simulink model "SEDC_Motor"  (R2023b)
settings: Solver=VariableStepAuto  StartTime=0.0  StopTime=0.1  MaxStep=1e-4  RelTol=1e-3
libraries: spsThyristorLib x4, spsVoltageMeasurementLib x3, spsACVoltageSourceLib x1, dspswit3 x1, spsSeriesRLCBranchLib x1, spsUniversalBridgeLib x1, sps_lib x1
settings Model: Creator=SEIF  LastModifiedBy=SEIF

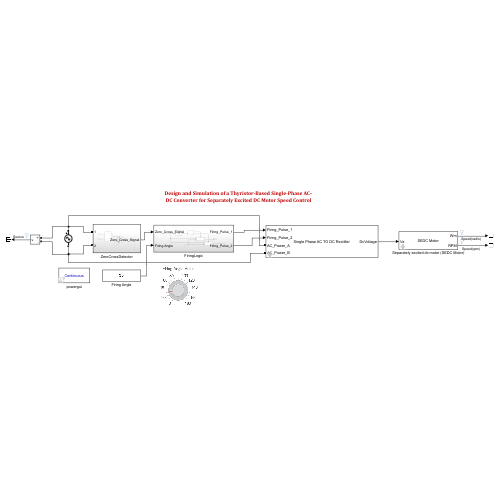
[thumbnail: Simulink's stored preview of the top-level diagram]
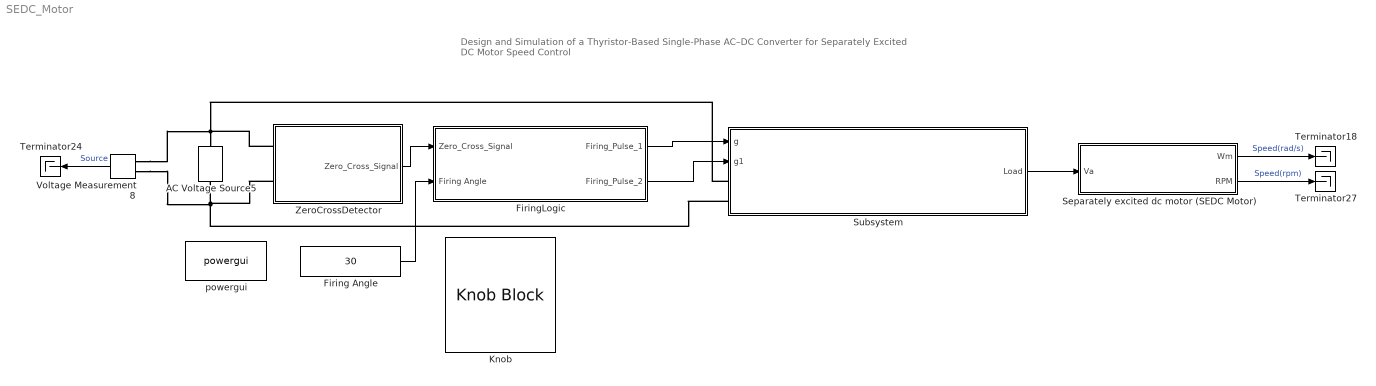
== system SEDC_Motor ==
  note: Design and Simulation of a Thyristor-Based Single-Phase AC–DC Converter for Separately Excited DC Motor Speed Control
  AC Voltage Source5 : spsACVoltageSourceLib/AC Voltage Source  Amplitude=sqrt(2) * 220  Phase=0  Frequency=50  SampleTime=0  Measurements=None  BusType=swing  Pref=10e3  Qref=0  Qmin=-inf  Qmax=+inf
  Firing Angle : Constant  Value=30
  FiringLogic : Subsystem
  Knob : KnobBlock  ScaleMax=180
  Separately excited dc motor (SEDC Motor) : Subsystem  mask{Ra=50, La=0.15, J=0.05, B=0.005, Kt=1.15, Kphi=1.15, TL=5}
      mask prompts: Ra "Armature Resistance"; La "Armature Inductance"; J "Moment of Inertia"; B "Viscous Friction"; Kt "Torque Constant"; Kphi "Back EMF Constant"; TL "Load Torque"
      mask Display:
      | disp('SEDC Motor');
      | 
      | port_label('input',1,'Va');
      | port_label('output',1,'Wm');
      | port_label('output',2,'RPM');
  Subsystem : Subsystem
      mask Display:
      | disp('Single Phase AC TO DC Rectifier');
      | 
      | port_label('input',1,'Firing_Pulse_1');
      | port_label('input',2,'Firing_Pulse_2');
      | port_label('lconn',1,'AC_Power_A');
      | port_label('lconn',2,'AC_Power_B');
      | port_label('output',1,'DcVoltage');
  Terminator18 : Terminator
  Terminator24 : Terminator
  Terminator27 : Terminator
  Voltage Measurement8 : spsVoltageMeasurementLib/Voltage Measurement  PhasorSimulation=off  OutputType=Complex  PSBequivalent=0
  ZeroCrossDetector : Subsystem
  powergui : sps_lib/powergui  Priority=1  SimulationMode=Continuous  SampleTime=50e-6  frequency=60  Iterations=50  frequencyindice=50  Pbase=100e6  ErrMax=1e-4  UnitsV=kV  UnitsW=MW  buscounter=0  FunctionMessages=off  echomessages=off  EnableUseOfTLC=off  CurrentSourceSwitches=off  DisableSnubberDevices=off  DisableRonSwitches=off  DisableVfSwitches=off  DisplayEquations=off  AutomaticDiscreteSolvers=off  SolverType=Tustin/Backward Euler (TBE)  Interpol=off  ExternalGateDelay=off  methode=off  Ts=100  x0status=blocks  SPID=on  SwTol=0  HookPort=off  NonlinearTolerance=1e-4  nMaxIteration=100  ContinueOnMaxIteration=off  RestoreLinks=warning  ResistiveCurrentMeasurement=off  Frange=[0:2:500]  Ylog=off  Xlog=on  ShowGrid=off  save=off  variable=ZData  structure=0  ZoomFFT=off  StartTime=0.0  cycles=1  DisplayStyle=1  fundamental=60  FreqAxis=off  MaxFrequency=1000  frequencyindicesteady=1  RmsSteady=1  display=off
  wires:
  Separately excited dc motor (SEDC Motor)/1(Wm) -> Terminator18/1  "Speed(rad/s)"
  ZeroCrossDetector/1(Zero_Cross_Signal) -> FiringLogic/1(Zero_Cross_Signal)
  Separately excited dc motor (SEDC Motor)/2(RPM) -> Terminator27/1  "Speed(rpm)"
  Voltage Measurement8/1 -> Terminator24/1  "Source"
  Firing Angle/1 -> FiringLogic/2(Firing Angle)
  Subsystem/1(Load) -> Separately excited dc motor (SEDC Motor)/1(Va)
  FiringLogic/1(Firing_Pulse_1) -> Subsystem/1(g)
  FiringLogic/2(Firing_Pulse_2) -> Subsystem/2(g1)
  connections:
  Voltage Measurement8/LConn2 -- Subsystem/LConn2 -- ZeroCrossDetector/LConn2 -- AC Voltage Source5/LConn1
  Voltage Measurement8/LConn1 -- Subsystem/LConn1 -- ZeroCrossDetector/LConn1 -- AC Voltage Source5/RConn1

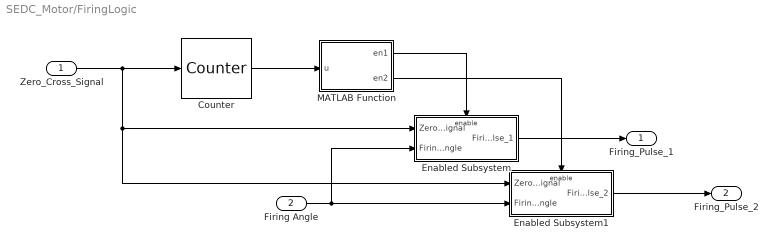
== system SEDC_Motor/FiringLogic ==
  Zero_Cross_Signal : Inport
  Firing Angle : Inport  Port=2
  Counter : dspswit3/Counter  Direction=Up  CountEvent=Rising edge  CounterSize=User defined  MaxCount=255  InitialCount=0  Output=Count  HitValue=32  ResetInput=off  SamplesPerFrame=1  Ts=1  CntDtype=double  HitDtype=Logical
  Enabled Subsystem : Subsystem  TreatAsAtomicUnit=on
  Enabled Subsystem1 : Subsystem  TreatAsAtomicUnit=on
  MATLAB Function : MATLAB Function  TreatAsAtomicUnit=on
  Firing_Pulse_1 : Outport
  Firing_Pulse_2 : Outport  Port=2
  wires:
  Zero_Cross_Signal/1 -> Enabled Subsystem1/1(Zero_Cross_Signal), Enabled Subsystem/1(Zero_Cross_Signal), Counter/1
  Counter/1 -> MATLAB Function/1(u)
  Firing Angle/1 -> Enabled Subsystem1/2(Firing Angle), Enabled Subsystem/2(Firing Angle)
  Enabled Subsystem/1(Firing_Pulse_1) -> Firing_Pulse_1/1
  Enabled Subsystem1/1(Firing_Pulse_2) -> Firing_Pulse_2/1
  MATLAB Function/1(en1) -> Enabled Subsystem/Enable
  MATLAB Function/2(en2) -> Enabled Subsystem1/Enable

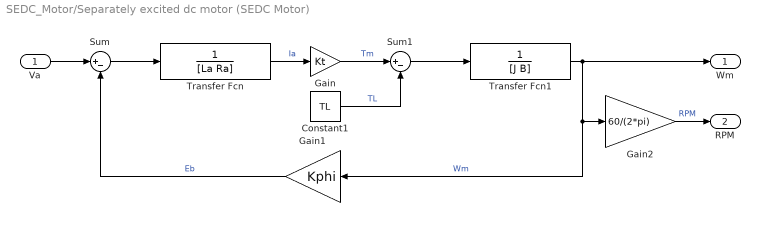
== system SEDC_Motor/Separately excited dc motor (SEDC Motor) ==
  Va : Inport
  Constant1 : Constant  Value=TL
  Gain : Gain  Gain=Kt
  Gain1 : Gain  Gain=Kphi
  Gain2 : Gain  Gain=60/(2*pi)
  Sum : Sum  Inputs=|+-
  Sum1 : Sum  Inputs=|+-
  Transfer Fcn : TransferFcn  Denominator=[La Ra]
  Transfer Fcn1 : TransferFcn  Denominator=[J B]
  Wm : Outport
  RPM : Outport  Port=2
  wires:
  Sum/1 -> Transfer Fcn/1
  Va/1 -> Sum/1
  Gain1/1 -> Sum/2  "Eb"
  Transfer Fcn/1 -> Gain/1  "Ia"
  Gain/1 -> Sum1/1  "Tm"
  Constant1/1 -> Sum1/2  "TL"
  Sum1/1 -> Transfer Fcn1/1
  Transfer Fcn1/1 -> Gain1/1, Gain2/1, Wm/1  "Wm"
  Gain2/1 -> RPM/1  "RPM"

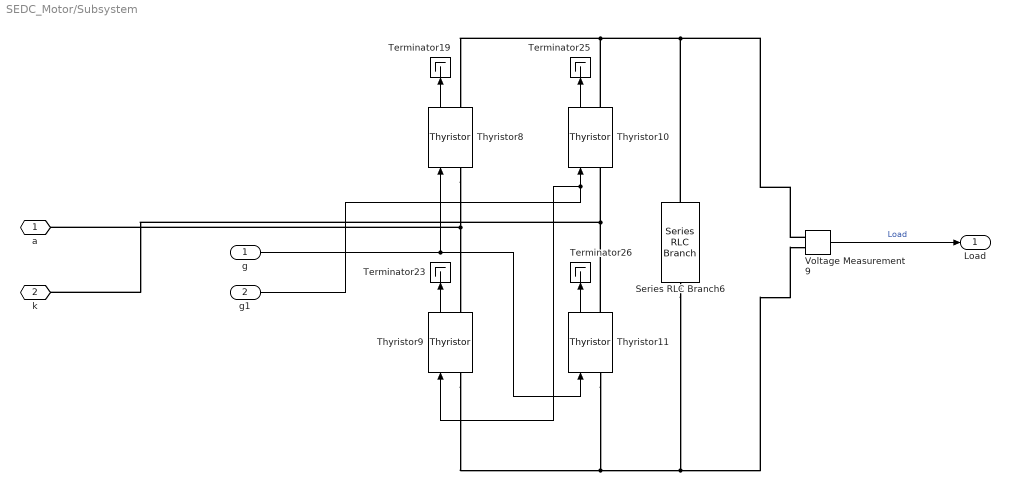
== system SEDC_Motor/Subsystem ==
  g : Inport
  g1 : Inport  Port=2
  Series RLC Branch6 : spsSeriesRLCBranchLib/Series RLC Branch  LConnTagsString=__new0  RConnTagsString=__new0  BranchType=C  Resistance=50  Inductance=1e-3  SetiL0=off  InitialCurrent=0  Capacitance=1  Setx0=off  InitialVoltage=0  Measurements=None
  Terminator{19,23,25..26} (4 alike) : Terminator
  Thyristor{8..11} (4 alike) : spsThyristorLib/Thyristor  Ron=0.001  Lon=0  Vf=0.8  IC=0  Rs=500  Cs=250e-9  Measurements=on
  Voltage Measurement9 : spsVoltageMeasurementLib/Voltage Measurement  PhasorSimulation=off  OutputType=Complex  PSBequivalent=0
  a : PMIOPort  Side=Left
  k : PMIOPort  Port=2  Side=Left
  Load : Outport
  wires:
  Thyristor11/1 -> Terminator26/1
  Thyristor8/1 -> Terminator19/1
  g1/1 -> Thyristor9/1, Thyristor10/1
  Thyristor9/1 -> Terminator23/1
  Thyristor10/1 -> Terminator25/1
  Voltage Measurement9/1 -> Load/1  "Load"
  g/1 -> Thyristor11/1, Thyristor8/1
  connections:
  Thyristor9/LConn1 -- Thyristor11/LConn1 -- Voltage Measurement9/LConn2 -- Series RLC Branch6/RConn1
  Thyristor8/LConn1 -- Thyristor9/RConn1 -- a/RConn1
  Thyristor10/LConn1 -- Thyristor11/RConn1 -- k/RConn1
  Series RLC Branch6/LConn1 -- Voltage Measurement9/LConn1 -- Thyristor8/RConn1 -- Thyristor10/RConn1

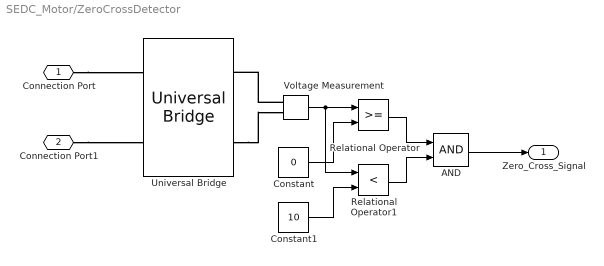
== system SEDC_Motor/ZeroCrossDetector ==
  AND : Logic  AllPortsSameDT=off  OutDataTypeStr=boolean
  Constant : Constant  Value=0
  Constant1 : Constant  Value=10
  Relational Operator : RelationalOperator  OutDataTypeStr=boolean  RndMeth=Simplest  InputSameDT=off
  Relational Operator1 : RelationalOperator  Operator=<  OutDataTypeStr=boolean  RndMeth=Simplest  InputSameDT=off
  Universal Bridge : spsUniversalBridgeLib/Universal Bridge  Arms=2  SnubberResistance=1e5  SnubberCapacitance=inf  Device=Diodes  Ron=1e-3  Lon=0  ForwardVoltages="[  0  0  ]"  ForwardVoltage=0  GTOparameters=[ 10e-6 , 20e-6 ]  IGBTparameters=[ 1e-6 , 2e-6 ]  Measurements=None  Measurements_2=None  converterType=Rectifier
  Voltage Measurement : spsVoltageMeasurementLib/Voltage Measurement  PhasorSimulation=off  OutputType=Complex  PSBequivalent=0
  Connection Port : PMIOPort  Side=Left
  Connection Port1 : PMIOPort  Port=2  Side=Left
  Zero_Cross_Signal : Outport
  wires:
  Voltage Measurement/1 -> Relational Operator1/1, Relational Operator/1
  Constant/1 -> Relational Operator/2
  Constant1/1 -> Relational Operator1/2
  Relational Operator/1 -> AND/1
  Relational Operator1/1 -> AND/2
  AND/1 -> Zero_Cross_Signal/1
  connections:
  Connection Port/RConn1 -- Universal Bridge/LConn1
  Connection Port1/RConn1 -- Universal Bridge/LConn2
  Voltage Measurement/LConn1 -- Universal Bridge/RConn1
  Universal Bridge/RConn2 -- Voltage Measurement/LConn2

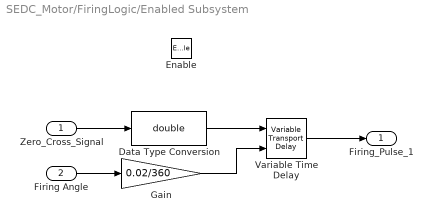
== system SEDC_Motor/FiringLogic/Enabled Subsystem ==
  Zero_Cross_Signal : Inport
  Firing Angle : Inport  Port=2
  Enable : EnablePort
  Data Type Conversion : DataTypeConversion  OutDataTypeStr=double  SaturateOnIntegerOverflow=off  RndMeth=Floor
  Gain : Gain  Gain=0.02/360
  Variable Time Delay : VariableTransportDelay  MaximumDelay=10
  Firing_Pulse_1 : Outport
  wires:
  Zero_Cross_Signal/1 -> Data Type Conversion/1
  Firing Angle/1 -> Gain/1
  Gain/1 -> Variable Time Delay/2
  Variable Time Delay/1 -> Firing_Pulse_1/1
  Data Type Conversion/1 -> Variable Time Delay/1

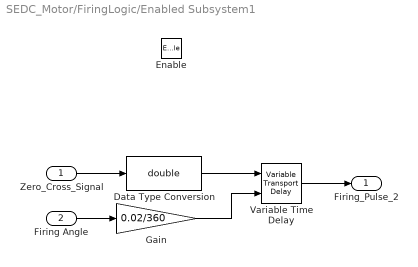
== system SEDC_Motor/FiringLogic/Enabled Subsystem1 ==
  Zero_Cross_Signal : Inport
  Firing Angle : Inport  Port=2
  Enable : EnablePort
  Data Type Conversion : DataTypeConversion  OutDataTypeStr=double  SaturateOnIntegerOverflow=off  RndMeth=Floor
  Gain : Gain  Gain=0.02/360
  Variable Time Delay : VariableTransportDelay  MaximumDelay=10
  Firing_Pulse_2 : Outport
  wires:
  Firing Angle/1 -> Gain/1
  Gain/1 -> Variable Time Delay/2
  Variable Time Delay/1 -> Firing_Pulse_2/1
  Data Type Conversion/1 -> Variable Time Delay/1
  Zero_Cross_Signal/1 -> Data Type Conversion/1

== matlab function SEDC_Motor/FiringLogic/MATLAB Function ==
  data: u input; en1 output; en2 output
function [en1, en2] = fcn(u)

en1 = 0;
en2 = 0;


if mod(u, 2) == 0
    en1 = 1;
    en2 = 0;
end

if mod(u, 2) == 1
    en1 = 0;
    en2 = 1;
end
